simulink model "pranav_plant_iteration1"  (R2025a)
settings: Solver=VariableStepAuto  StartTime=0.0  StopTime=10.0  RelTol=1e-3
libraries: simulink_extras x1
settings Model: Creator=kuppa  LastModifiedBy=kuppa

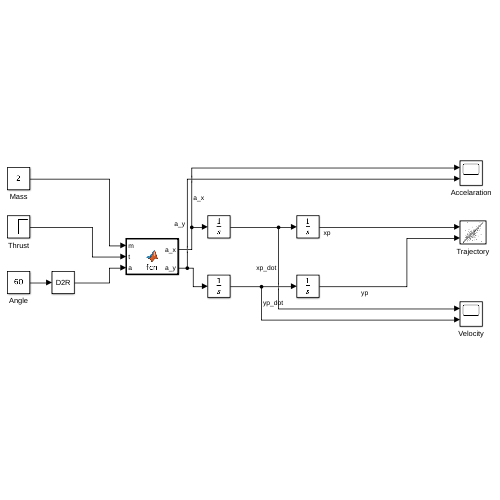
[thumbnail: Simulink's stored preview of the top-level diagram]
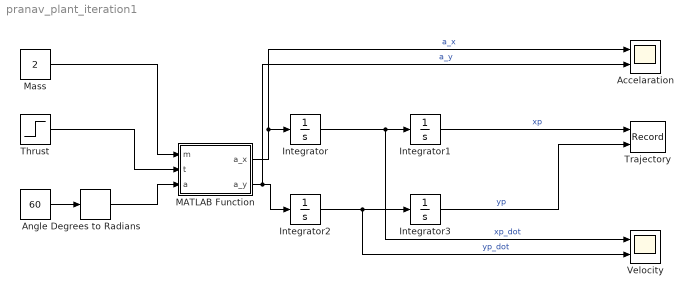
== system pranav_plant_iteration1 ==
  Accelaration : Scope  NumInputPorts=2
      settings: ActiveDisplayYMinimum=-2.1929508291370796  ActiveDisplayYMaximum=1.9649055296856588
  Angle : Constant  Value=60
  Degrees to Radians : simulink_extras/Transformations/Degrees to Radians
  Integrator : Integrator
  Integrator1 : Integrator
  Integrator2 : Integrator
  Integrator3 : Integrator  InitialCondition=100
  MATLAB Function : MATLAB Function  TreatAsAtomicUnit=on
  Mass : Constant  Value=2
  Thrust : Step  After=30  SampleTime=0
  Trajectory : Record  NumPorts=2.0  FileSettingsInternal="{\"entries\":[{\"content\":{\"excelSettings\":{\"content\":{},\"type\":\"Streamout.ExcelSettings\"},\"parquetSettings\":{\"content\":{},\"type\":\"Streamout.ParquetSettings\"}},\"type\":\"Streamout.FileSettingStorage\",\"uuid\":\"\"}],\"packageUris\":[\"http:\\/\\/schema.mathworks.com\\/mf0\\/streamout_blocks\\/R2020a\"],\"version\":\"1.0\"}"  FrameSettings=[0, 0]  Layout=[1 1]  SignalsInternal="{\"entries\":[{\"content\":{\"signals\":[{\"content\":{\"blockPath\":[],\"dimensions\":[1],\"domain\":\"\",\"lineColor\":\"#a2142f\",\"plots\":[ 1 ],\"port\":1,\"sid\":[\"\"],\"signalID\":1,\"signalName\":\"xp\"},\"type\":\"RecordBlkView.Signal\",\"uuid\":\"\"},{\"content\":{\"blockPath\":[],\"dimensions\":[1],\"domain\":\"\",\"lineColor\":\"#139fff\",\"plots\":[ 1 ],\"port\":2,\"sid\":[\"\"],\"signalID\":2,\"signalName\":\"yp\"},\"type\":\"RecordBlkView.Signal\",\"uuid\":\"\"}]},\"type\":\"RecordBlkView.InputSignals\",\"uuid\":\"\"}],\"packageUris\":[\"http:\\/\\/schema.mathworks.com\\/mf0\\/streamout_blocks\\/R2020a\"],\"version\":\"1.0\"}"  VisualizationBindings="{\"xyplotplugin\":{\"info\":[{\"series\":[{\"bindingParametersList\":[{\"parameter\":\"X-Axis\",\"signalID\":1,\"signalName\":\"xp\"},{\"parameter\":\"Y-Axis\",\"signalID\":2,\"signalName\":\"yp\"}],\"seriesID\":0}],\"subplotID\":1}]}}"  CompatibilityTag=XY
  Velocity : Scope  NumInputPorts=2
      settings: ActiveDisplayYMinimum=-19.473750000000003  ActiveDisplayYMaximum=77.163750000000007
  wires:
  Angle/1 -> Degrees to Radians/1
  Degrees to Radians/1 -> MATLAB Function/3(a)
  Thrust/1 -> MATLAB Function/2(t)
  Mass/1 -> MATLAB Function/1(m)
  Integrator/1 -> Velocity/1, Integrator1/1  "xp_dot"
  MATLAB Function/1(a_x) -> Accelaration/1, Integrator/1  "a_x"
  Integrator2/1 -> Velocity/2, Integrator3/1  "yp_dot"
  MATLAB Function/2(a_y) -> Accelaration/2, Integrator2/1  "a_y"
  Integrator1/1 -> Trajectory/1  "xp"
  Integrator3/1 -> Trajectory/2  "yp"

== matlab function pranav_plant_iteration1/MATLAB Function ==
  data: m input; t input; a input; a_x output; a_y output
function [a_x,a_y]= fcn(m, t, a)

g = 9.81;
a_x = (t*cos(a))/m;
a_y = (t*sin(a))/m - g;
